simulink model "scheme_L2"  (R2025b)
settings: Solver=VariableStepAuto  StartTime=0.0  StopTime=10.0  RelTol=1e-3
settings Model: Creator=sahan  LastModifiedBy=sahan

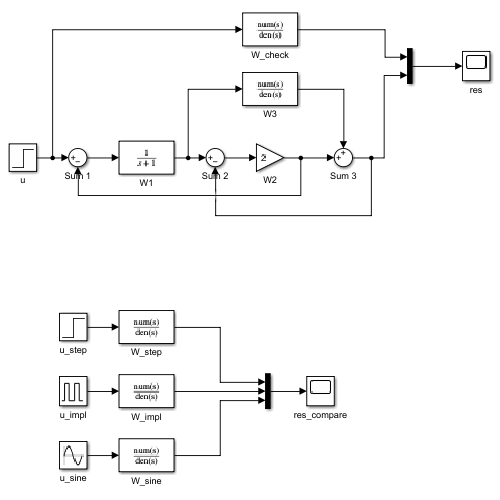
[thumbnail: Simulink's stored preview of the top-level diagram]
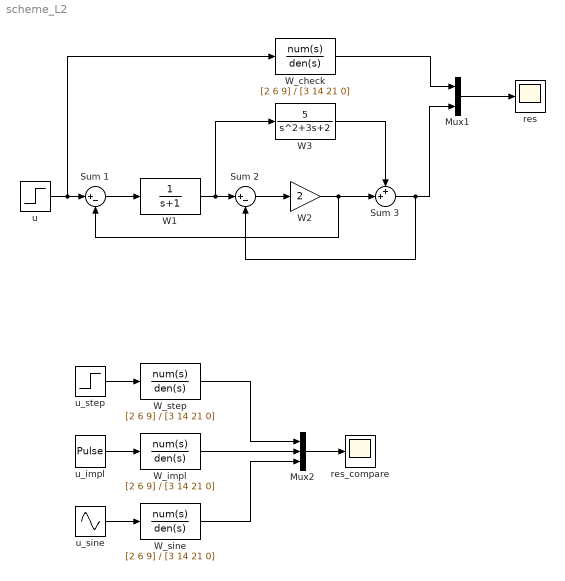
== system scheme_L2 ==
  Mux1 : Mux  Inputs=2
  Mux2 : Mux  Inputs=3
  Sum 1 : Sum  Inputs=|+-
  Sum 2 : Sum  Inputs=|+-
  Sum 3 : Sum  Inputs=++|
  W1 : TransferFcn  Denominator=[1 1]
  W2 : Gain  Gain=2
  W3 : TransferFcn  Numerator=[5]  Denominator=[1 3 2]
  W_check : TransferFcn  Numerator=[2 6 9]  Denominator=[3 14 21 0]
  W_impl : TransferFcn  Numerator=[2 6 9]  Denominator=[3 14 21 0]
  W_sine : TransferFcn  Numerator=[2 6 9]  Denominator=[3 14 21 0]
  W_step : TransferFcn  Numerator=[2 6 9]  Denominator=[3 14 21 0]
  res : Scope
      settings: ActiveDisplayYMinimum=-0.4821428571252474  ActiveDisplayYMaximum=4.3392857141272279
  res_compare : Scope
      settings: ActiveDisplayYMinimum=-0.4821428571252474  ActiveDisplayYMaximum=4.3392857141272279
  u : Step  SampleTime=0
  u_impl : DiscretePulseGenerator  PulseType=Time based  Period=10  PulseWidth=5
  u_sine : Sin  SampleTime=0
  u_step : Step  SampleTime=0
  wires:
  u/1 -> W_check/1, Sum 1/1
  Sum 1/1 -> W1/1
  W1/1 -> W3/1, Sum 2/1
  Sum 2/1 -> W2/1
  W3/1 -> Sum 3/1
  W2/1 -> Sum 3/2, Sum 1/2
  Sum 3/1 -> Sum 2/2, Mux1/2
  Mux1/1 -> res/1
  W_check/1 -> Mux1/1
  u_step/1 -> W_step/1
  W_sine/1 -> Mux2/3
  Mux2/1 -> res_compare/1
  W_impl/1 -> Mux2/2
  u_sine/1 -> W_sine/1
  W_step/1 -> Mux2/1
  u_impl/1 -> W_impl/1
